simulink model "solar_mppt_subsystem"  (R2026a)
settings: Solver=FixedStepAuto  StopTime=1
values from neighbouring files (symbols this model uses):
  irradiance_day = pchip(t_coarse, irradiance_coarse, t_sim)    [flc_init.m]
  t_sim = linspace(0, 1.0, 1001)    [flc_init.m]
undefined symbols (not defined in the file or in its folder): DiscIntNeverNeededParam
libraries: nesl_utility x5, fl_lib x4, ee_lib x2, fuzblock x1, eePwmGenerator x1
settings Model: Creator=user  LastModifiedBy=user

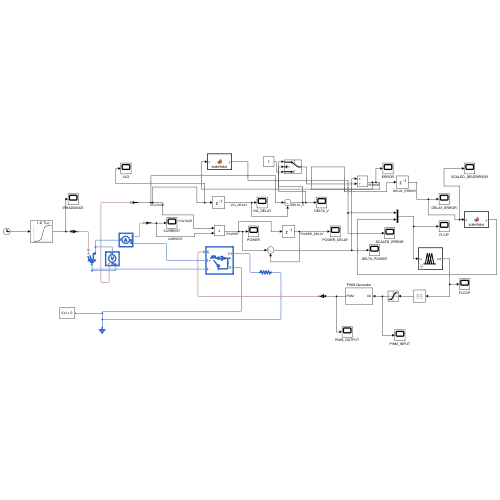
[thumbnail: Simulink's stored preview of the top-level diagram]
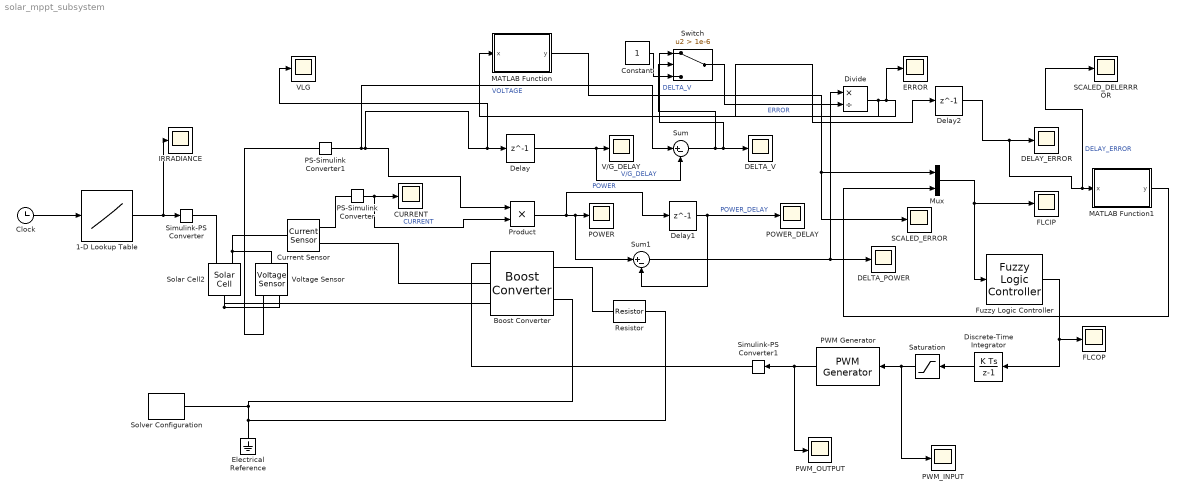
== system solar_mppt_subsystem ==
  1-D Lookup Table : Lookup_n-D  NumberOfTableDimensions=1  BreakpointsForDimension1=t_sim  Table=irradiance_day  ExtrapMethod=Clip  InternalRulePriority=Speed  RndMeth=Simplest
  Boost Converter : ee_lib/Semiconductors & Converters/Converters/Boost Converter  port_option=ee.enum.controlport.ps  device_type=ee.enum.converters.switchingdevice.ideal  Vf=0.8 V  Ron=0.001 Ohm  Rds=0.001 Ohm  Goff=1e-5 1/Ohm  Vgt=1 V  Vgt_off=-1 V  Ih=1 A  Vth=6 V  K=0  diode_param=ee.enum.converters.protectiondiode.nodynamics  diode_Vf=0.8 V  diode_Ron=0.001 Ohm  diode_Goff=1e-5 1/Ohm  diode_C=50 nF  diode_iRM=-235 A  diode_iF=300 A  diode_idot=-50 A/us  diode_trr_param=ee.enum.converters.diodetrr.trr_factor  diode_trr_factor=3  diode_trr=15 us  diode_Qrr=1500 s*uA  Lf=1e-6 H  Rl=0 Ohm  Cf=1e-7 F  Rf=1e-6 Ohm  snubber_type=ee.enum.converters.snubber.exclude  Cs=1e-7 F  Rs=0.1 Ohm  iL_specify=off  iL_priority=High  iL=0 A  iL_nominal_specify=off  iL_nominal_value=1  iL_nominal_unit=A  vc_specify=off  vc_priority=High  vc=0 V  vc_nominal_specify=off  vc_nominal_value=1  vc_nominal_unit=V
  CURRENT : Scope
      settings: ActiveDisplayYMinimum=-0.41351020650465781  ActiveDisplayYMaximum=3.7215920776010369
  Clock : Clock
  Constant : Constant
  Current Sensor : fl_lib/Electrical/Electrical Sensors/Current Sensor
  DELAY_ERROR : Scope
      settings: ActiveDisplayYMinimum=-0.932438052271241  ActiveDisplayYMaximum=7.5437756032088767  DataLoggingVariableName=ScopeData8
  DELTA_POWER : Scope
      settings: DataLoggingVariableName=ScopeData6
  DELTA_V : Scope
      settings: ActiveDisplayYMinimum=-1  ActiveDisplayYMaximum=1  DataLoggingVariableName=ScopeData3
  Delay : Delay  DelayLength=1  InitialCondition=0  InputProcessing=Columns as channels (frame based)
  Delay1 : Delay  DelayLength=1  InitialCondition=0  InputProcessing=Columns as channels (frame based)
  Delay2 : Delay  DelayLength=1  InitialCondition=0  InputProcessing=Columns as channels (frame based)
  Discrete-Time Integrator : DiscreteIntegrator  InitialCondition=0.4  SampleTime=-1  ICPrevOutput=DiscIntNeverNeededParam  ICPrevScaledInput=DiscIntNeverNeededParam
  Divide : Product  Inputs=*/
  ERROR : Scope
      settings: ActiveDisplayYMinimum=-0.932438052271241  ActiveDisplayYMaximum=7.5437756032088767  DataLoggingVariableName=ScopeData7
  Electrical Reference : fl_lib/Electrical/Electrical Elements/Electrical Reference
  FLCIP : Scope
      settings: ActiveDisplayYMinimum=-0.932438052271241  ActiveDisplayYMaximum=7.5437756032088767  DataLoggingVariableName=ScopeData10
  FLCOP : Scope
      settings: ActiveDisplayYMinimum=-1  ActiveDisplayYMaximum=1  DataLoggingVariableName=ScopeData9
  Fuzzy Logic Controller : fuzblock/Fuzzy Logic  Controller  FIS=mppt_fuzzy  OutputSampleNumber=101  DataType=double  UseLookupTable=off  NumBreakpoints=10  FuzzifiedInputs=off  RuleFiringStrengths=off  RuleOutputs=off  AggregatedOutputs=off  SimulateUsing=Interpreted execution  OutOfRangeInputValueMessage=warning  NoRuleFiredMessage=warning  EmptyOutputFuzzySetMessage=warning
  IRRADIANCE : Scope
      settings: ActiveDisplayYMinimum=-124.88690159999997  ActiveDisplayYMaximum=1124.9821144  DataLoggingVariableName=ScopeData16
  MATLAB Function : MATLAB Function  TreatAsAtomicUnit=on
  MATLAB Function1 : MATLAB Function  TreatAsAtomicUnit=on
  Mux : Mux  Inputs=2
  POWER : Scope
      settings: ActiveDisplayYMinimum=-14.008630460713221  ActiveDisplayYMaximum=126.07767894526859  DataLoggingVariableName=ScopeData4
  POWER_DELAY : Scope
      settings: Title=Output Power  ActiveDisplayYMinimum=-14.008630460713221  ActiveDisplayYMaximum=126.07767894526859  YLabel=Power Po(in watts)  DataLoggingVariableName=Po  DataLoggingSaveFormat=Array
  PS-Simulink Converter : nesl_utility/PS-Simulink Converter  PhysicalDomain=network_engine_domain  SubClassName=ps_output  LeftPortType=input  RightPortType=output  PseudoPeriodic=off  Frequencies=[]  VectorFormat=inherit  Unit=inherit  AffineConversion=off
  PS-Simulink Converter1 : nesl_utility/PS-Simulink Converter  PhysicalDomain=network_engine_domain  SubClassName=ps_output  LeftPortType=input  RightPortType=output  PseudoPeriodic=off  Frequencies=[]  VectorFormat=inherit  Unit=inherit  AffineConversion=off
  PWM Generator : eePwmGenerator/PWM Generator  CarrCount=Up  Tper=0.001  Tdelay=0  Ts=5e-5
  PWM_INPUT : Scope
      settings: ActiveDisplayYMinimum=-1  ActiveDisplayYMaximum=1  DataLoggingVariableName=ScopeData12
  PWM_OUTPUT : Scope
      settings: ActiveDisplayYMinimum=-1  ActiveDisplayYMaximum=1  DataLoggingVariableName=ScopeData11
  Product : Product
  Resistor : fl_lib/Electrical/Electrical Elements/Resistor  R=10 Ohm  i_specify=off  i_priority=None  i=0 A  i_nominal_specify=off  i_nominal_value=1  i_nominal_unit=A  v_specify=off  v_priority=None  v=0 V  v_nominal_specify=off  v_nominal_value=1  v_nominal_unit=V
  SCALED_DELERRROR : Scope
      settings: ActiveDisplayYMinimum=-1  ActiveDisplayYMaximum=1  DataLoggingVariableName=ScopeData14
  SCALED_ERROR : Scope
      settings: ActiveDisplayYMinimum=-1  ActiveDisplayYMaximum=1  DataLoggingVariableName=ScopeData13
  Saturation : Saturate  UpperLimit=0.9  LowerLimit=0.05
  Simulink-PS Converter : nesl_utility/Simulink-PS Converter  PhysicalDomain=network_engine_domain  SubClassName=ps_input  LeftPortType=input  RightPortType=output  PseudoPeriodic=off  Frequencies=[]  NoiseDistribution=none  NoiseParameters=[]  Unit=1  AffineConversion=off  FilteringAndDerivatives=provide  SimscapeFilterOrder=1  InputFilterTimeConstant=0.001  UdotUserProvided=0
  Simulink-PS Converter1 : nesl_utility/Simulink-PS Converter  PhysicalDomain=network_engine_domain  SubClassName=ps_input  LeftPortType=input  RightPortType=output  PseudoPeriodic=off  Frequencies=[]  NoiseDistribution=none  NoiseParameters=[]  Unit=1  AffineConversion=off  FilteringAndDerivatives=provide  SimscapeFilterOrder=1  InputFilterTimeConstant=0.001  UdotUserProvided=0
  Solar Cell2 : ee_lib/Sources/Solar Cell  prm=ee.enum.sources.solar_cell_prm.eightParameter  Isc=7.34 A  Voc=21.5 V  Is=1e-10 A  Is2=1e-10 A  Iph=7.34 A  Ir0=1000 W/m^2  ec=1.5  N2=2  Rs=0 Ohm  Rp=inf Ohm  N_series=36  N_parallel=1  TIPH1=0 1/K  EG=1.11 eV  TXIS1=3  TXIS2=3  TRS1=0  TRP1=0  Tmeas=25 degC  TFIXED=25 degC  thermal_mass=100 J/K  initial_temperature=25 degC
  Solver Configuration : nesl_utility/Solver Configuration  PhysicalDomain=network_engine_domain  SubClassName=solver  LeftPortType=input  RightPortType=generic  Tones=[]  Harmonics=[]  SimulateNoise=off  Profile=off  UseLocalSampling=off  EnableSwitchedLinearOptims=on  FrequencyDomain=off  UseCCode=off  RelTol=0.001  AbsTol=0.001  MinStep=1e-09  ToWorkspace=off  RevertToSquareIcSolve=off  NumHomotopyIterations=100  PhasorMode=off  PhasorModeNumHarmonics=1  ConsistencySolver=NEWTON_XTOL_AFTER_FTOL  CanonicalOrdering=CANONICAL  OptimizeIntermediates=OPTIMIZED  IndexReductionMethod=DerivativeReplacement  DoDC=off  ResidualTolerance=1e-09  ConsistencyTolSource=GLOBAL  ConsistencyAbsTol=0.001  ConsistencyRelTol=0.001  ConsistencyTolFactor=0.001  UseLocalSolver=off  LocalSolverChoice=NE_BACKWARD_EULER_ADVANCER  ResolveIndetEquations=on  FunctionEvalNumThread=1  LocalSolverSampleTime=0.001  DoFixedCost=off  MaxNonlinIter=3  MaxModeIter=2  ComputeImpulses=off  ImpulseIterations=2  LinearAlgebra=auto  LinearAlgebraNumThread=0  EquationFormulation=NE_TIME_EF  DelaysMemoryBudget=1024  AutomaticFiltering=on  FilteringTimeConstant=0.001  PartitionStorageMethod=AS_NEEDED  PartitionMemoryBudget=1024  PartitionMethod=ROBUST  MultibodyUseLocalSolver=off  MultibodyLocalSolverChoice=ODE1  MultibodyLocalSolverSampleTime=0.001
  Sum : Sum  Inputs=|+-
  Sum1 : Sum  Inputs=|+-
  Switch : Switch  Criteria=u2 > Threshold  Threshold=1e-6  SaturateOnIntegerOverflow=off  InputSameDT=off
  V/G_DELAY : Scope
      settings: ActiveDisplayYMinimum=-3.3265921205731632  ActiveDisplayYMaximum=38.011121807218  DataLoggingVariableName=ScopeData2
  VLG : Scope
      settings: Title=Output Voltage  ActiveDisplayYMinimum=-3.3265921205731632  ActiveDisplayYMaximum=38.011121807218  YLabel=Solar output voltage(V)  DataLoggingVariableName=ScopeData15
  Voltage Sensor : fl_lib/Electrical/Electrical Sensors/Voltage Sensor
  wires:
  Clock/1 -> 1-D Lookup Table/1
  1-D Lookup Table/1 -> IRRADIANCE/1, Simulink-PS Converter/1
  PS-Simulink Converter1/1 -> Sum/1, VLG/1, Delay/1, Product/1  "VOLTAGE"
  Delay/1 -> Sum/2, V/G_DELAY/1  "V/G_DELAY"
  Sum/1 -> Switch/2, Switch/1, DELTA_V/1  "DELTA_V"
  PS-Simulink Converter/1 -> CURRENT/1, Product/2  "CURRENT"
  Product/1 -> Delay1/1, Sum1/1, POWER/1  "POWER"
  Delay1/1 -> Sum1/2, POWER_DELAY/1  "POWER_DELAY"
  Mux/1 -> FLCIP/1, Fuzzy Logic Controller/1
  Divide/1 -> MATLAB Function/1(x), Delay2/1, ERROR/1  "ERROR"
  Sum1/1 -> Divide/1, DELTA_POWER/1
  Delay2/1 -> SCALED_DELERRROR/1, MATLAB Function1/1(x), DELAY_ERROR/1  "DELAY_ERROR"
  Fuzzy Logic Controller/1 -> FLCOP/1, Discrete-Time Integrator/1
  Discrete-Time Integrator/1 -> Saturation/1
  Saturation/1 -> PWM_INPUT/1, PWM Generator/1
  PWM Generator/1 -> PWM_OUTPUT/1, Simulink-PS Converter1/1
  Constant/1 -> Switch/3
  Switch/1 -> Divide/2
  MATLAB Function1/1(y) -> Mux/2
  MATLAB Function/1(y) -> SCALED_ERROR/1, Mux/1
  connections:
  Simulink-PS Converter/RConn1 -- Solar Cell2/LConn1
  Solar Cell2/LConn2 -- Voltage Sensor/LConn1 -- Current Sensor/LConn1
  Current Sensor/RConn2 -- Boost Converter/LConn2
  Solar Cell2/RConn1 -- Boost Converter/LConn3 -- Voltage Sensor/RConn2
  Current Sensor/RConn1 -- PS-Simulink Converter/LConn1
  Voltage Sensor/RConn1 -- PS-Simulink Converter1/LConn1
  Simulink-PS Converter1/RConn1 -- Boost Converter/LConn1
  Electrical Reference/LConn1 -- Resistor/RConn1 -- Solver Configuration/RConn1 -- Boost Converter/RConn2
  Resistor/LConn1 -- Boost Converter/RConn1

== matlab function solar_mppt_subsystem/MATLAB Function ==
  data: x input; y output
function y = scaleValue(x)
    inMin = -0.5;
    inMax = 7.5;
    outMin = -1;
    outMax = 1;
    
    % Linear mapping
    scaled = outMin + ((x - inMin) / (inMax - inMin)) * (outMax - outMin);
    
    % Saturate the output between -1 and 1
    y = max(outMin, min(outMax, scaled));
end

== matlab function solar_mppt_subsystem/MATLAB Function1 ==
  data: x input; y output
function y = scaleValue(x)
    inMin = -0.5;
    inMax = 7.5;
    outMin = -1;
    outMax = 1;
    
    % Linear mapping
    scaled = outMin + ((x - inMin) / (inMax - inMin)) * (outMax - outMin);
    
    % Saturate the output between -1 and 1
    y = max(outMin, min(outMax, scaled));
end
